simulink model "TE6_model"  (R2026b)
settings: Solver=VariableStepAuto  StopTime=5
settings Model: Creator=User  LastModifiedBy=User

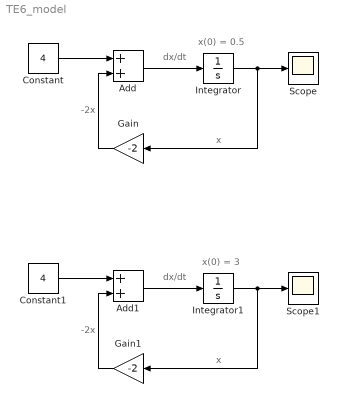
== system TE6_model ==
  note: x(0) = 3
  note: x(0) = 0.5
  note: x
  note: -2x
  note: dx/dt
  note: -2x
  note: dx/dt
  note: x
  Add : Sum
  Add1 : Sum
  Constant : Constant  Value=4
  Constant1 : Constant  Value=4
  Gain : Gain  Gain=-2
  Gain1 : Gain  Gain=-2
  Integrator : Integrator  InitialCondition=0.5
  Integrator1 : Integrator  InitialCondition=3
  Scope : Scope
      settings: ActiveDisplayYMinimum=0.31250851249716649  ActiveDisplayYMaximum=2.1874233875255022
  Scope1 : Scope
      settings: ActiveDisplayYMinimum=1.8750510749829981  ActiveDisplayYMaximum=3.124994325001889
  wires:
  Constant/1 -> Add/1
  Gain/1 -> Add/2
  Integrator/1 -> Scope/1, Gain/1
  Add/1 -> Integrator/1
  Constant1/1 -> Add1/1
  Gain1/1 -> Add1/2
  Add1/1 -> Integrator1/1
  Integrator1/1 -> Scope1/1, Gain1/1
